simulink model "Simulink_3_Control_Difuso_Motor_Arduino"  (R2023a)
settings: Solver=ode45  StartTime=0.0  StopTime=2.5  MaxStep=0.01  RelTol=1e-3
PreLoadFcn:
  | if ~exist('fis','var'), fis = readfis('ControlDifusoMotorDC.fis'); end
InitFcn:
  | if ~exist('fis','var'), fis = readfis('ControlDifusoMotorDC.fis'); end
libraries: fuzblock x1
settings Model: Creator=juanj  LastModifiedBy=juanj
settings RTWCC: GPUComputeCapability=5.0
settings ConfigComp: CovBoundaryAbsTol=1.0e-5

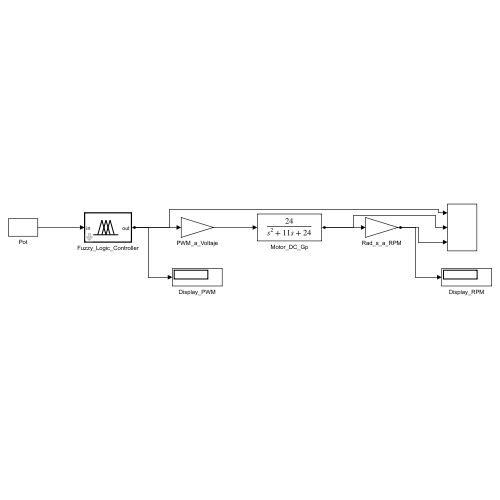
[thumbnail: Simulink's stored preview of the top-level diagram]
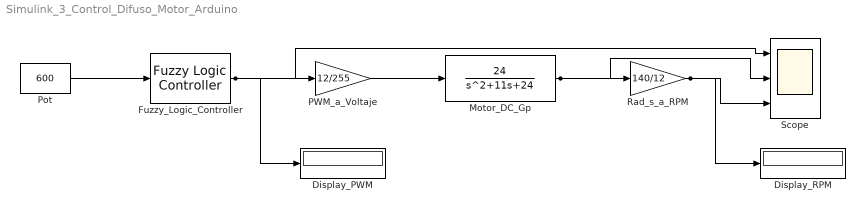
== system Simulink_3_Control_Difuso_Motor_Arduino ==
  Display_PWM : Display
  Display_RPM : Display
  Fuzzy_Logic_Controller : fuzblock/Fuzzy Logic  Controller  FIS=fis  OutputSampleNumber=101  DataType=double  FuzzifiedInputs=off  RuleFiringStrengths=off  RuleOutputs=off  AggregatedOutputs=off  SimulateUsing=Interpreted execution  OutOfRangeInputValueMessage=warning  NoRuleFiredMessage=warning  EmptyOutputFuzzySetMessage=warning
  Motor_DC_Gp : TransferFcn  Numerator=[24]  Denominator=[1 11 24]
  PWM_a_Voltaje : Gain  Gain=12/255
  Pot : Constant  Value=600
  Rad_s_a_RPM : Gain  Gain=140/12
  Scope : Scope  NumInputPorts=3
  wires:
  Pot/1 -> Fuzzy_Logic_Controller/1
  Fuzzy_Logic_Controller/1 -> PWM_a_Voltaje/1, Display_PWM/1, Scope/1
  PWM_a_Voltaje/1 -> Motor_DC_Gp/1
  Motor_DC_Gp/1 -> Rad_s_a_RPM/1, Scope/2
  Rad_s_a_RPM/1 -> Display_RPM/1, Scope/3
